simulink model "sf_timer_function_calls"  (R2025b)
settings: Solver=FixedStepDiscrete  StartTime=0.0  StopTime=10.0  FixedStep=1  RelTol=1e-3  EnableMultiTasking=on
libraries: sf_timer_utils_lib x2
settings Model: Creator=The MathWorks, Inc.  LastModifiedBy=The MathWorks, Inc.
settings SolverCC: AlgebraicLoopSolver=TrustRegion
settings DataIOCC: LimitDataPoints=on  SaveFormat=Array  ReturnWorkspaceOutputs=off
settings OptimizationCC: DefaultParameterBehavior=Inlined  ReuseModelBlockBuffer=off  ExpressionDepthLimit=2147483647.0  LifeSpan=inf
settings DebuggingCC: UnderspecifiedInitializationDetection=Classic  MergeDetectMultiDrivingBlocksExec=none  SolverPrmCheckMsg=warning  FcnCallInpInsideContextMsg=warning  UnconnectedInputMsg=warning  UnconnectedOutputMsg=warning  UnconnectedLineMsg=warning  StateNameClashWarn=warning  SFUnexpectedBacktrackingDiag=warning  SFNoUnconditionalDefaultTransitionDiag=warning  SFExecutionAtInitializationDiag=none  ArithmeticOperatorsInVariantConditions=warning
settings HardwareCC: ProdBitPerPointer=32.0  ProdBitPerSizeT=32.0  ProdBitPerPtrDiffT=32.0  ProdLargestAtomicFloat=None  ProdIntDivRoundTo=Undefined  ProdEndianess=Unspecified  ProdWordSize=32.0  ProdHWDeviceType=32-bit Generic
settings ModelReferenceCC: EnableRefExpFcnMdlSchedulingChecks=on  PropagateSignalLabelsOutOfModel=off
settings SFSimCC: SimUseLocalCustomCode=off
settings RTWCC: RTWUseLocalCustomCode=off  GPUComputeCapability=3.5  DLArmComputeVersion=19.05
settings CodeAppCC: StateflowObjectComments=on
settings GRTTargetCC: TargetLangStandard=C89/C90 (ANSI)  CombineOutputUpdateFcns=off  GRTInterface=on
settings ConfigComp: CovMetricSettings=dw  CovSaveCumulativeToWorkspaceVar=on  CovSaveSingleToWorkspaceVar=on  CovExternalEMLEnable=off

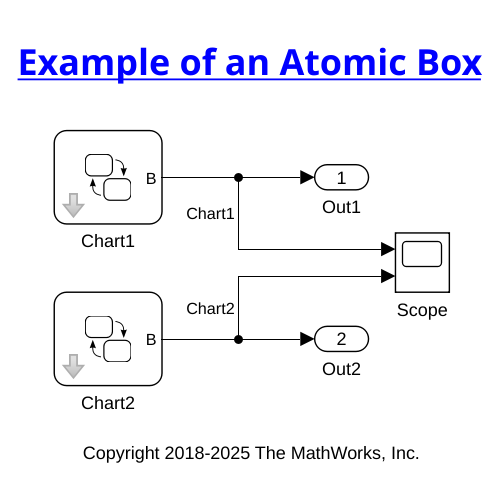
[thumbnail: Simulink's stored preview of the top-level diagram]
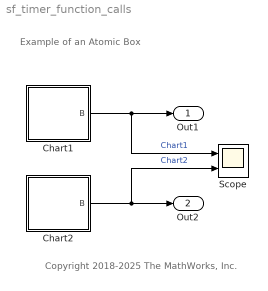
== system sf_timer_function_calls ==
  note: Copyright 2018-2025 The MathWorks, Inc.
  note: Example of an Atomic Box
  Chart1 : Stateflow chart  TreatAsAtomicUnit=on  mask{T=5}
      mask prompts: T "Threshold"
  Chart2 : Stateflow chart  TreatAsAtomicUnit=on  mask{T=7}
      mask prompts: T "Threshold"
  Scope : Scope  NumInputPorts=2
      settings: ActiveDisplayYMinimum=-0.125  ActiveDisplayYMaximum=1.125
  Out1 : Outport  VectorParamsAs1DForOutWhenUnconnected=off
  Out2 : Outport  Port=2  VectorParamsAs1DForOutWhenUnconnected=off
  wires:
  Chart1/1(" B") -> Out1/1, Scope/1  "Chart1"
  Chart2/1(" B") -> Out2/1, Scope/2  "Chart2"

== stateflow chart sf_timer_function_calls/Chart1 ==
  state A
    entry: t0 = Time.GetTime();
  state B
  state Time [group]
  (default) -> A
  A -> B : [Time.GetTime() - t0 >= T]
  data: t0 local double; B output boolean; T parameter

== stateflow chart sf_timer_function_calls/Chart2 ==
  state A
    entry: t0 = Time.GetTime();
  state B
  state Time [group]
  (default) -> A
  A -> B : [Time.GetTime() - t0 >= T]
  data: t0 local double; T parameter; B output boolean
